simulink model "PAMESA_ExerciseOnSimulink"  (R2026a)
settings: Solver=VariableStepAuto  StopTime=0
settings Model: Creator=Dawn  LastModifiedBy=Dawn

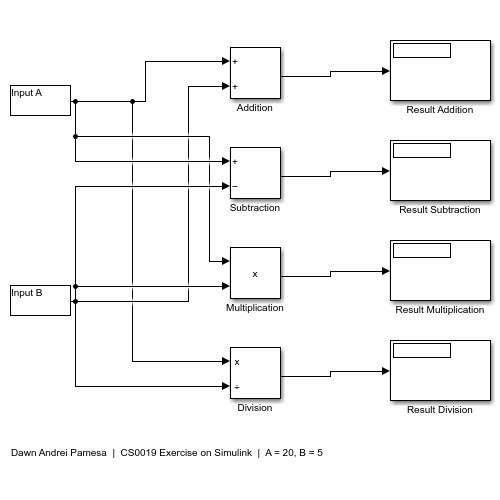
[thumbnail: Simulink's stored preview of the top-level diagram]
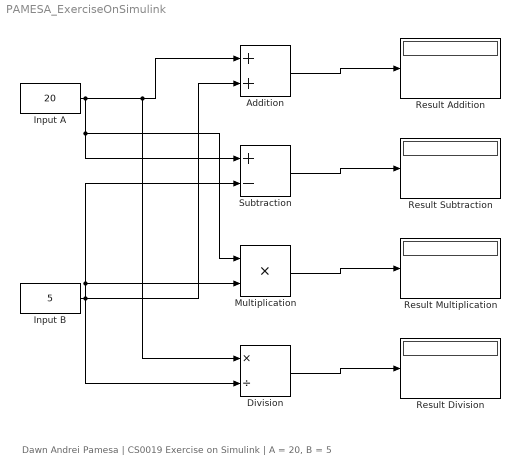
== system PAMESA_ExerciseOnSimulink ==
  note: Dawn Andrei Pamesa | CS0019 Exercise on Simulink | A = 20, B = 5
  Addition : Sum
  Division : Product  Inputs=*/
  Input A : Constant  Value=20
  Input B : Constant  Value=5
  Multiplication : Product  Inputs=**
  Result Addition : Display
  Result Division : Display
  Result Multiplication : Display
  Result Subtraction : Display
  Subtraction : Sum  Inputs=+-
  wires:
  Input A/1 -> Addition/1, Division/1, Subtraction/1, Multiplication/1
  Input B/1 -> Subtraction/2, Multiplication/2, Addition/2, Division/2
  Addition/1 -> Result Addition/1
  Subtraction/1 -> Result Subtraction/1
  Multiplication/1 -> Result Multiplication/1
  Division/1 -> Result Division/1
